simulink model "ekf_orbit_sim"  (R2025b)
settings: Solver=ode4  StartTime=0.0  StopTime=sim_param.t_final  FixedStep=sim_param.dt_sim  RelTol=1e-3
undefined symbols (not defined in the file): C_nm, P0, Q, R, S_nm, sim_param, x_hat_0, x_true_0
settings Model: Creator=Lenovo  LastModifiedBy=Lenovo
settings DataIOCC: ReturnWorkspaceOutputs=off

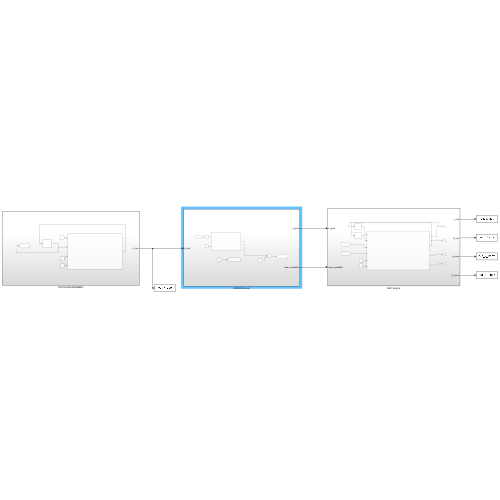
[thumbnail: Simulink's stored preview of the top-level diagram]
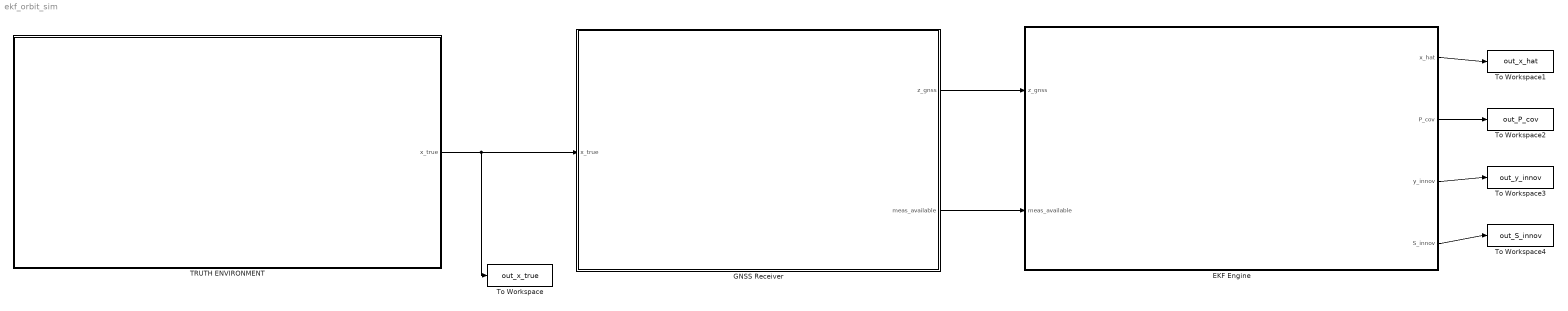
== system ekf_orbit_sim ==
  EKF Engine : Subsystem
  GNSS Receiver : Subsystem
  TRUTH ENVIRONMENT : Subsystem
  To Workspace : ToWorkspace  VariableName=out_x_true  SaveFormat=Timeseries  SampleTime=-1
  To Workspace1 : ToWorkspace  VariableName=out_x_hat  SaveFormat=Timeseries  SampleTime=-1
  To Workspace2 : ToWorkspace  VariableName=out_P_cov  SaveFormat=Timeseries  SampleTime=-1
  To Workspace3 : ToWorkspace  VariableName=out_y_innov  SaveFormat=Timeseries  SampleTime=-1
  To Workspace4 : ToWorkspace  VariableName=out_S_innov  SaveFormat=Timeseries  SampleTime=-1
  wires:
  TRUTH ENVIRONMENT/1(x_true) -> To Workspace/1, GNSS Receiver/1(x_true)
  GNSS Receiver/1(z_gnss) -> EKF Engine/1(z_gnss)
  GNSS Receiver/2(meas_available) -> EKF Engine/2(meas_available)
  EKF Engine/1(x_hat) -> To Workspace1/1
  EKF Engine/2(P_cov) -> To Workspace2/1
  EKF Engine/3(y_innov) -> To Workspace3/1
  EKF Engine/4(S_innov) -> To Workspace4/1

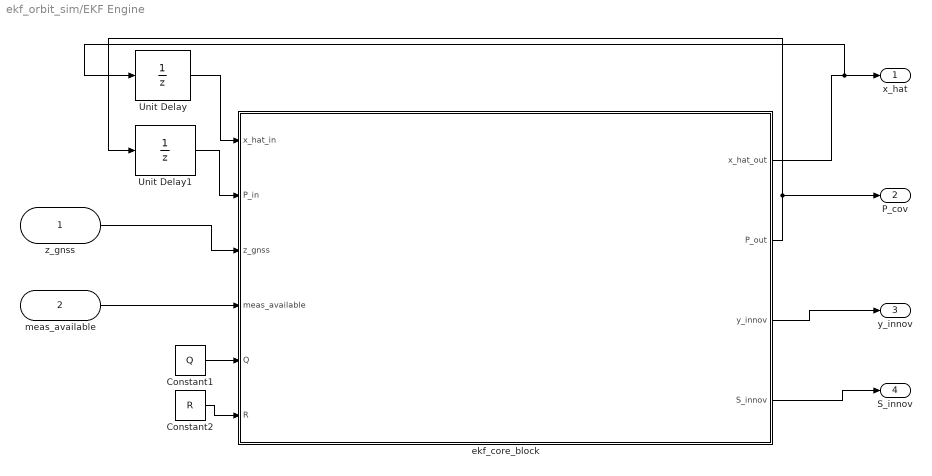
== system ekf_orbit_sim/EKF Engine ==
  z_gnss : Inport
  meas_available : Inport  Port=2
  Constant1 : Constant  Value=Q
  Constant2 : Constant  Value=R
  Unit Delay : UnitDelay  InitialCondition=x_hat_0  SampleTime=sim_param.dt_sim  HasFrameUpgradeWarning=on
  Unit Delay1 : UnitDelay  InitialCondition=P0  SampleTime=sim_param.dt_sim  HasFrameUpgradeWarning=on
  ekf_core_block : MATLAB Function  TreatAsAtomicUnit=on
  x_hat : Outport
  P_cov : Outport  Port=2
  y_innov : Outport  Port=3
  S_innov : Outport  Port=4
  wires:
  Unit Delay/1 -> ekf_core_block/1(x_hat_in)
  Unit Delay1/1 -> ekf_core_block/2(P_in)
  Constant1/1 -> ekf_core_block/5(Q)
  Constant2/1 -> ekf_core_block/6(R)
  z_gnss/1 -> ekf_core_block/3(z_gnss)
  meas_available/1 -> ekf_core_block/4(meas_available)
  ekf_core_block/2(P_out) -> P_cov/1, Unit Delay1/1
  ekf_core_block/3(y_innov) -> y_innov/1
  ekf_core_block/4(S_innov) -> S_innov/1
  ekf_core_block/1(x_hat_out) -> Unit Delay/1, x_hat/1

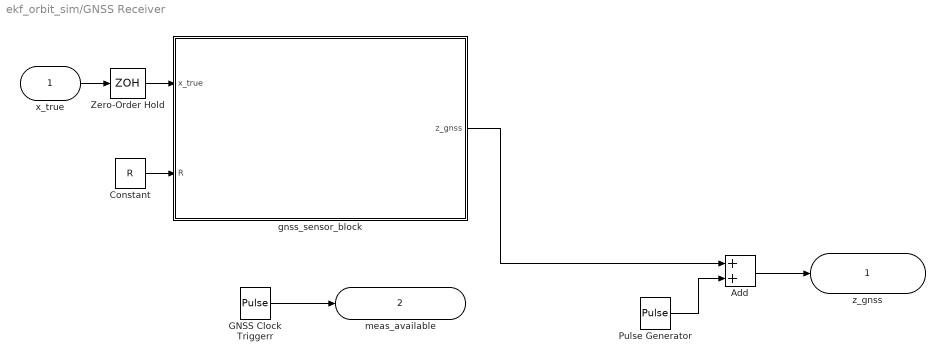
== system ekf_orbit_sim/GNSS Receiver ==
  x_true : Inport
  Add : Sum
  Constant : Constant  Value=R
  GNSS Clock Triggerr : DiscretePulseGenerator  PulseType=Time based  Period=1.0  PulseWidth=10  PhaseDelay=1.0
  Pulse Generator : DiscretePulseGenerator  PulseType=Time based  Amplitude=[500; 500; 500; 0; 0; 0]  Period=20000  PulseWidth=0.005  PhaseDelay=3000
  Zero-Order Hold : ZeroOrderHold  SampleTime=1.0
  gnss_sensor_block : MATLAB Function  TreatAsAtomicUnit=on
  z_gnss : Outport
  meas_available : Outport  Port=2
  wires:
  Constant/1 -> gnss_sensor_block/2(R)
  Zero-Order Hold/1 -> gnss_sensor_block/1(x_true)
  x_true/1 -> Zero-Order Hold/1
  gnss_sensor_block/1(z_gnss) -> Add/1
  GNSS Clock Triggerr/1 -> meas_available/1
  Add/1 -> z_gnss/1
  Pulse Generator/1 -> Add/2

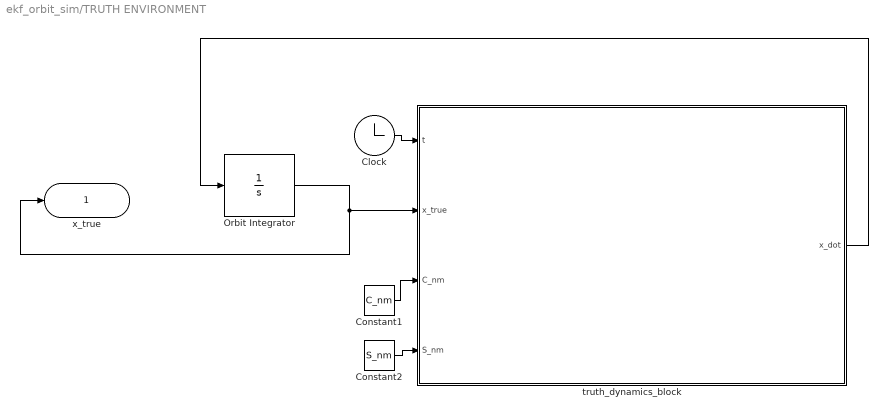
== system ekf_orbit_sim/TRUTH ENVIRONMENT ==
  Clock : Clock
  Constant1 : Constant  Value=C_nm
  Constant2 : Constant  Value=S_nm
  Orbit Integrator : Integrator  InitialCondition=x_true_0
  truth_dynamics_block : MATLAB Function  TreatAsAtomicUnit=on
  x_true : Outport
  wires:
  Clock/1 -> truth_dynamics_block/1(t)
  Constant2/1 -> truth_dynamics_block/4(S_nm)
  Constant1/1 -> truth_dynamics_block/3(C_nm)
  Orbit Integrator/1 -> x_true/1, truth_dynamics_block/2(x_true)
  truth_dynamics_block/1(x_dot) -> Orbit Integrator/1

== matlab function ekf_orbit_sim/GNSS Receiver/gnss_sensor_block ==
  data: x_true input; z_gnss output; R input
function z_gnss = gnss_sensor_block(x_true, R)
    z_gnss = gnss_sensor_model(x_true, R);
end

== matlab function ekf_orbit_sim/TRUTH ENVIRONMENT/truth_dynamics_block ==
  data: t input; x_dot output; x_true input; C_nm input; S_nm input; sim_param parameter
function x_dot = truth_dynamics_block(t, x_true, C_nm, S_nm, sim_param)
    x_dot = truth_dynamics(t, x_true, sim_param, C_nm, S_nm);
end

== matlab function ekf_orbit_sim/EKF Engine/ekf_core_block ==
  data: x_hat_in input; x_hat_out output; P_in input; z_gnss input; meas_available input; Q input; R input; P_out output; y_innov output; S_innov output; sim_param parameter
function [x_hat_out, P_out, y_innov, S_innov] = ekf_core_block(x_hat_in, P_in, z_gnss, meas_available, Q, R, sim_param)
    [x_hat_out, P_out, y_innov, S_innov] = ekf_predict_update(x_hat_in, P_in, z_gnss, meas_available, sim_param, Q, R);
end
